simulink model "HoMoLapVehicle"  (R2024b)
settings: Solver=FixedStepDiscrete  StartTime=0.0  StopTime=165  FixedStep=1/600  RelTol=1e-3
model workspace (MAT data in the model file):
  HL.C.L = 1.53
  HL.C.tf = 1.24
  HL.C.tr = 1.2
  HL.C.Fz0 = 600
  HL.C.rr = 0.015
  HL.C.rho = 1.225
  HL.C.eta = 0.97
  HL.C.R = 0.202
  HL.C.C = 1.4
  HL.C.m = 252
  HL.C.b = 0.765
  HL.C.a = 0.765
  HL.C.h = 0.293
  HL.C.Iz = 135
  HL.C.mu0 = 1.4
  HL.C.muExp = -0.1
  HL.C.ap = 0.12217304764
  HL.C.B = 16.9965588703
  HL.C.Pmax = 80000
  HL.C.Tm = 21
  HL.C.G = 12.421
  HL.C.nmax = 20000
  HL.C.brakeFront = 0.7
  HL.C.Fb = 9000
  HL.C.rollFront = 0.65
  HL.C.tv = 1
  HL.C.delMax = 0.436332312999
  HL.C.ClA = 5.4
  HL.C.CdA = 1.7
  HL.C.bal = 0.5
  HL.C.vMotor = 34.0606884054
  HL.C.FdMax = 5010.21326733
  HL.C.yawLoss = 0.0115
  HL.C.arc.grip = 1.18
  HL.C.arc.power = 1.75
  HL.C.arc.force = 1.2
  HL.C.arc.vtop = 1.45
  HL.C.arc.grass = 0.85
  HL.C.arc.brake = 1.35
  HL.P.N = 1104
  HL.P.K = [0.00557564962824 0.00557192851623 0.00444398359644 0.00333258349506 0.00444242884758 0.00444161481707 0.00665900821826 0.00665501835401 0.00775978966829 0.00449481541894 0.00227428503847 5.56249943769e-05 ... (1104 elements, 1104x1)]
  HL.P.vPlan = [30.1075218866 39.1055718469 38.5151228391 37.927644757 37.3430291371 36.761078832 36.1817671084 35.6048349068 35.0303058287 34.4576046366 33.8870589928 33.3185370499 ... (1104 elements, 1104x1)]
  HL.P.vPlanA = [31.7069851745 41.4425106581 40.7940160778 40.1494163588 39.5085862113 38.8713036493 38.2375335601 37.6069871673 36.9796848558 36.3549943319 35.7332682213 35.1143579177 ... (1104 elements, 1104x1)]
  HL.P.world = [-5 -5 307.7 185.75]
  HL.T.N = 1104
  HL.T.x = [103.24 104.24 105.24 106.24 107.24 108.24 109.24 110.24 111.24 112.24 113.24 114.24 ... (1104 elements, 1104x1)]
  HL.T.y = [54.28 54.28 54.29 54.3 54.31 54.33 54.35 54.38 54.41 54.46 54.51 54.56 ... (1104 elements, 1104x1)]
  HL.T.SEG = [1 1.00004999875 1.00004999875 1.00004999875 1.00019998 1.00019998 1.0004498988 1.0004498988 1.00124921973 1.00124921973 1.00124921973 0.991261822124 ... (1104 elements, 1104x1)]
  HL.T.S = [0 1 2.00004999875 3.0000999975 4.00014999625 5.00034997625 6.00054995626 7.00099985505 8.00144975385 9.00269897357 10.0039481933 11.005197413 ... (1105 elements, 1105x1)]
  HL.T.LEN = 1103.39618369
  HL.T.TTX = [0.999987500234 0.999987500234 0.99995000375 0.99995000375 0.999887518981 0.99980005998 0.999687646408 0.999550303522 0.999200958722 0.998752338878 0.998752338878 0.998739791817 ... (1104 elements, 1104x1)]
  HL.T.TTY = [-0.00499993750117 0.00499993750117 0.00999950003749 0.0099995000375 0.0149983127847 0.0199960011996 0.0249921911602 0.0299865091057 0.0399680383489 0.0499376169439 0.0499376169439 0.050187929237 ... (1104 elements, 1104x1)]
  HL.T.NX = [0.00499993750117 -0.00499993750117 -0.00999950003749 -0.0099995000375 -0.0149983127847 -0.0199960011996 -0.0249921911602 -0.0299865091057 -0.0399680383489 -0.0499376169439 -0.0499376169439 -0.050187929237 ... (1104 elements, 1104x1)]
  HL.T.NY = [0.999987500234 0.999987500234 0.99995000375 0.99995000375 0.999887518981 0.99980005998 0.999687646408 0.999550303522 0.999200958722 0.998752338878 0.998752338878 0.998739791817 ... (1104 elements, 1104x1)]
  HL.T.K = [0.00557564962824 0.00557192851623 0.00444398359644 0.00333258349506 0.00444242884758 0.00444161481707 0.00665900821826 0.00665501835401 0.00775978966829 0.00449481541894 0.00227428503847 5.56249943769e-05 ... (1104 elements, 1104x1)]
  HL.T.APRON = [26 26 276.7 154.75]
  HL.c0.x = 105.269947697
  HL.c0.y = 42.9591015691
  HL.c0.h = 3.12159531962
  HL.c0.vx = 0
  HL.c0.vy = 0
  HL.c0.r = 0
  HL.c0.st = 0
  HL.c0.thr = 0
  HL.c0.brk = 0
  HL.c0.delta = 0
  HL.c0.axp = 0
  HL.c0.ayp = 0
  HL.c0.s = 1073.39618369
  HL.c0.lat = 0
  HL.c0.grass = 0
  HL.c0.driftT = 0
  HL.c0.dLim = 0.4
  HL.c0.assistBrake = 0
  HL.c0.outT = 0
  HL.c0.hitWall = 0
  HL.c0.FyfP = 0
  HL.c0.FyrP = 0
  HL.arcade = 0
  HL.dt = 0.00166666666667
  HL.lts.s = [0 1.99997495707 3.99994991414 5.99992487121 7.99989982828 9.99987478535 11.9998497424 13.9998246995 15.9997996566 17.9997746136 19.9997495707 21.9997245278 ... (552 elements, 552x1)]
  HL.lts.t = [0 0.13 0.249 0.359 0.462 0.558 0.65 0.737 0.82 0.901 0.979 1.056 ... (552 elements, 552x1)]
  HL.lts.v = [14.62 16.11 17.51 18.84 20.1 21.32 22.46 23.47 24.37 25.18 25.93 26.62 ... (552 elements, 552x1)]
  HL.lts.lapTime = 75.058
Description:
  | HoMo-LAP: FAUmax tau single-track model with the AI driver on the FSG endurance track (generated by build_homolap_model.m).
settings Model: Creator=Archit  LastModifiedBy=Archit

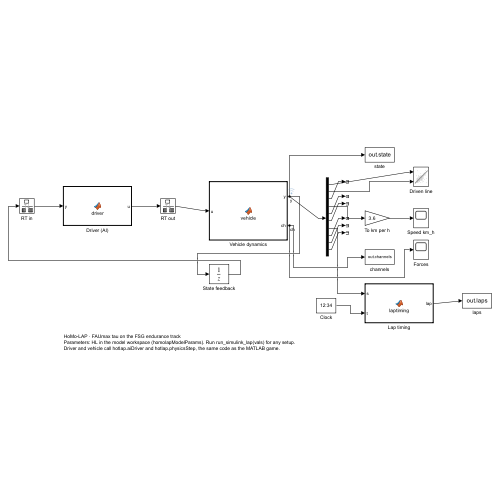
[thumbnail: Simulink's stored preview of the top-level diagram]
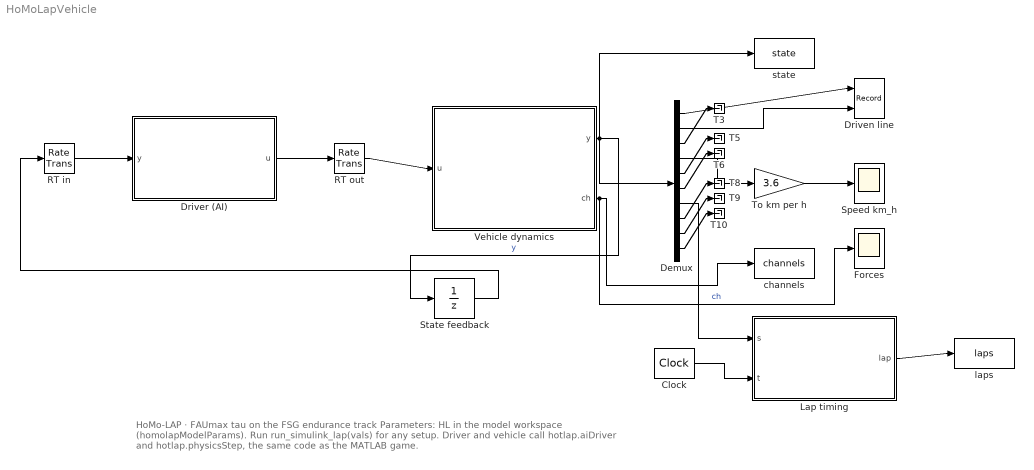
== system HoMoLapVehicle ==
  note: HoMo-LAP · FAUmax tau on the FSG endurance track
      | Parameters: HL in the model workspace (homolapModelParams). Run run_simulink_lap(vals) for any setup.
      | Driver and vehicle call hotlap.aiDriver and hotlap.physicsStep, the same code as the MATLAB game.
  Clock : DigitalClock  SampleTime=1/600
  Demux : Demux  Outputs=10
  Driven line : Record  FileSettingsInternal="{\"entries\":[{\"content\":{\"excelSettings\":{\"content\":{},\"type\":\"Streamout.ExcelSettings\"}},\"type\":\"Streamout.FileSettingStorage\",\"uuid\":\"\"}],\"packageUris\":[\"http:\\/\\/schema.mathworks.com\\/mf0\\/streamout_blocks\\/R2020a\"],\"version\":\"1.0\"}"  Layout=[1 1]  SignalsInternal="{\"entries\":[{\"content\":{\"signals\":[{\"content\":{\"blockPath\":[],\"dimensions\":[1],\"domain\":\"\",\"lineColor\":\"#a2142f\",\"plots\":[ 1 ],\"port\":1,\"signalID\":1,\"signalName\":\"XY Graph:1\"},\"type\":\"RecordBlkView.Signal\",\"uuid\":\"\"},{\"content\":{\"blockPath\":[],\"dimensions\":[1],\"domain\":\"\",\"lineColor\":\"#139fff\",\"plots\":[ 1 ],\"port\":2,\"signalID\":2,\"signalName\":\"XY Graph:2\"},\"type\":\"RecordBlkView.Signal\",\"uuid\":\"\"}]},\"type\":\"RecordBlkView.InputSignals\",\"uuid\":\"\"}],\"packageUris\":[\"http:\\/\\/schema.mathworks.com\\/mf0\\/streamout_blocks\\/R2020a\"],\"version\":\"1.0\"}"  VisualizationBindings="{\"xyplotplugin\":{\"info\":[{\"series\":[{\"bindingParametersList\":[{\"parameter\":\"X-Axis\",\"signalID\":1,\"signalName\":\"XY Graph:1\"},{\"parameter\":\"Y-Axis\",\"signalID\":2,\"signalName\":\"XY Graph:2\"}],\"seriesID\":0}],\"subplotID\":1}]}}"  CompatibilityTag=XY
  Driver (AI) : MATLAB Function  TreatAsAtomicUnit=on
  Forces : Scope
  Lap timing : MATLAB Function  TreatAsAtomicUnit=on
  RT in : RateTransition  OutPortSampleTime=4/600
  RT out : RateTransition  OutPortSampleTime=1/600
  Speed km_h : Scope
  State feedback : UnitDelay  InitialCondition=zeros(10,1)  SampleTime=1/600  HasFrameUpgradeWarning=on
  T{3,5..6,8..10} (6 alike) : Terminator
  To km per h : Gain  Gain=3.6
  Vehicle dynamics : MATLAB Function  TreatAsAtomicUnit=on
  channels : ToWorkspace  VariableName=channels  SaveFormat=Timeseries  SampleTime=-1
  laps : ToWorkspace  VariableName=laps  SaveFormat=Timeseries  SampleTime=-1
  state : ToWorkspace  VariableName=state  SaveFormat=Timeseries  SampleTime=-1
  wires:
  State feedback/1 -> RT in/1
  RT in/1 -> Driver (AI)/1(y)
  Driver (AI)/1(u) -> RT out/1
  RT out/1 -> Vehicle dynamics/1(u)
  Vehicle dynamics/1(y) -> State feedback/1, Demux/1, state/1  "y"
  Vehicle dynamics/2(ch) -> channels/1, Forces/1  "ch"
  Demux/1 -> Driven line/1
  Demux/2 -> Driven line/2
  Demux/4 -> To km per h/1
  To km per h/1 -> Speed km_h/1
  Demux/7 -> Lap timing/1(s)
  Clock/1 -> Lap timing/2(t)
  Lap timing/1(lap) -> laps/1
  Demux/3 -> T3/1
  Demux/5 -> T5/1
  Demux/6 -> T6/1
  Demux/8 -> T8/1
  Demux/9 -> T9/1
  Demux/10 -> T10/1

== matlab function HoMoLapVehicle/Driver (AI) ==
  data: y input; u output; HL parameter
function u = driver(y, HL)
% AI driver (hotlap.aiDriver): curvature feed-forward, heading and cross-track correction, speed plan.
% y = [x y h vx vy r s lat dLim delta] from the vehicle; u = [steer thr brk].
c = struct('x', y(1), 'y', y(2), 'h', y(3), 'vx', y(4), 'vy', y(5), 's', y(7), 'lat', y(8), 'dLim', max(y(9), 0.05));
inp = hotlap.aiDriver(c, HL.T, HL.P.vPlan);
u = [inp.steer; inp.thr; inp.brk];

== matlab function HoMoLapVehicle/Lap timing ==
  data: s input; lap output; t input; HL parameter
function lap = laptiming(s, t, HL)
% Lap counter at the start/finish line (s wraps from the lap length to 0); lap = [count last lap time].
persistent prev t0 n last
if isempty(prev), prev = s; t0 = -1; n = 0; last = 0; end
L = HL.T.LEN; d = s - prev;
if d < -L / 2
    d = d + L; tc = t - (s / max(d, 1e-6)) * (4 / 600);
    if t0 >= 0, n = n + 1; last = tc - t0; end
    t0 = tc;
end
prev = s;
lap = [n; last];

== matlab function HoMoLapVehicle/Vehicle dynamics ==
  data: u input; y output; ch output; HL parameter
function [y, ch] = vehicle(u, HL)
% Single-track model (hotlap.physicsStep) at 600 Hz, lap position every 4 steps as in the game.
% y = [x y h vx vy r s lat dLim delta]; ch = [Fdown Fdrag ax ay P beta grip_g].
persistent c k
if isempty(c), c = HL.c0; k = 0; end
inp = hotlap.driverInput(u(1), u(2), u(3), false, false, false, HL.arcade);
[c, f] = hotlap.physicsStep(c, inp, HL.C, HL.P, HL.dt);
k = k + 1;
if mod(k, 4) == 0
    nr = hotlap.nearestPoint(HL.T, c.x, c.y); c.s = nr.s; c.lat = nr.lat;
    a = HL.T.APRON; c.grass = ~(c.x > a(1) && c.x < a(3) && c.y > a(2) && c.y < a(4));
end
y = [c.x; c.y; c.h; c.vx; c.vy; c.r; c.s; c.lat; c.dLim; c.delta];
ch = [f.Fdown; f.Fdrag; f.ax; f.ay; f.P; f.beta; (f.capF + f.capR) / (HL.C.m * 9.81)];
